simulink model "ghe3_ik_reference"  (Simulink 8.9)
settings: Solver=ode4  SolverType=Fixed-step  StopTime=22.2222222222  FixedStep=0.01
undefined symbols (not defined in the file or in its folder): ghe3_reference_ik, ghe3_reference_parameters

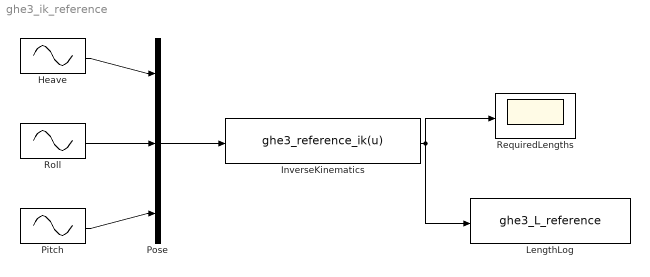
== system ghe3_ik_reference ==
  Heave : Sin  Amplitude=.02  Bias=ghe3_reference_parameters.h0  Frequency=2*pi*.09  Phase=0  SampleTime=0
  Roll : Sin  Amplitude=4*pi/180  Bias=0  Frequency=2*pi*.09  Phase=pi/2  SampleTime=0
  Pitch : Sin  Amplitude=4*pi/180  Bias=0  Frequency=2*pi*.09  Phase=0  SampleTime=0
  Pose : Mux  Inputs=3
  InverseKinematics : MATLABFcn  MATLABFcn=ghe3_reference_ik(u)  OutputDimensions=3
  RequiredLengths : Scope
  LengthLog : ToWorkspace  VariableName=ghe3_L_reference  SaveFormat=Structure With Time
  wires:
  Heave/1 -> Pose/1
  Roll/1 -> Pose/2
  Pitch/1 -> Pose/3
  Pose/1 -> InverseKinematics/1
  InverseKinematics/1 -> RequiredLengths/1, LengthLog/1
